simulink model "nape_speed_brakes"  (R2024b)
settings: Solver=VariableStepAuto  StartTime=0.0  StopTime=t_fin  RelTol=1e-3
InitFcn:
  | setup_speed_brakes
values from neighbouring files (symbols this model uses):
  alpha0L = convang(-2.9,'deg','rad')    [setup_speed_brakes.m]
  alphabMax = convang(8.0,'deg','rad')    [setup_speed_brakes.m]
  CD0 = 0.020    (= 0.02)    [setup_speed_brakes.m]
  delta0 = convang(0.0,'deg','rad')    [setup_speed_brakes.m]
  deltac = convang(15,'deg','rad')    [setup_speed_brakes.m]
  deltac2 = convang(15,'deg','rad')    [setup_speed_brakes.m]
  deltac3 = convang(0,'deg','rad')    [setup_speed_brakes.m]
  deltac4 = convang(0,'deg','rad')    [setup_speed_brakes.m]
  g = 9.81    [setup_speed_brakes.m]
  gamma0 = convang(0.0,'deg','rad')    [setup_speed_brakes.m]
  gammac = convang(5,'deg','rad')    [setup_speed_brakes.m]
  gammac2 = convang(0,'deg','rad')    [setup_speed_brakes.m]
  gammac3 = convang(-5,'deg','rad')    [setup_speed_brakes.m]
  gammac4 = convang(0,'deg','rad')    [setup_speed_brakes.m]
  h0 = 3048    [setup_speed_brakes.m]
  kD1 = 2/(S*pi*AReffective)    (= 0.000338404785343)    [setup_speed_brakes.m]
  kL = 2/(S*CLalpha)    (= 0.0012483552919)    [setup_speed_brakes.m]
  kLI = 0.010    (= 0.01)    [setup_speed_brakes.m]
  kLP = 0.50    (= 0.5)    [setup_speed_brakes.m]
  kLSB = -0.00008    (= -8e-05)    [setup_speed_brakes.m]
  knu = 0.075    [setup_speed_brakes.m]
  kSB = -0.00008    (= -8e-05)    [setup_speed_brakes.m]
  kTI = 0.0020    (= 0.002)    [setup_speed_brakes.m]
  kTP = 0.080    (= 0.08)    [setup_speed_brakes.m]
  kWdot = 1.31*1e-5    (= 1.31e-05)    [setup_speed_brakes.m]
  L0 = weight0*cos(gamma0)*cos(nu0)    [setup_speed_brakes.m]
  mass0 = massNom    (= 129003)    [setup_speed_brakes.m]
  nu0 = convang(0.0,'deg','rad')    [setup_speed_brakes.m]
  pL = 2.50    (= 2.5)    [setup_speed_brakes.m]
  pnu = 1.00    (= 1)    [setup_speed_brakes.m]
  pT = 2.00    (= 2)    [setup_speed_brakes.m]
  S = 279.6    [setup_speed_brakes.m]
  SB_AlphaFactorMax = 4    [setup_speed_brakes.m]
  SB_AlphaGain = 0.01    [setup_speed_brakes.m]
  SB_DragFactorMax = 1.5    [setup_speed_brakes.m]
  T0 = D0 + weight0*sin(gamma0)    [setup_speed_brakes.m]
  tc = 5    [setup_speed_brakes.m]
  tc2 = 90    [setup_speed_brakes.m]
  tc3 = 150    [setup_speed_brakes.m]
  tc4 = 240    [setup_speed_brakes.m]
  TMax = 320272    [setup_speed_brakes.m]
  V0 = 178.8    [setup_speed_brakes.m]
  Vc = convvel(450,'mph','m/s')    [setup_speed_brakes.m]
  Vc2 = convvel(420,'mph','m/s')    [setup_speed_brakes.m]
  Vc3 = convvel(400,'mph','m/s')    [setup_speed_brakes.m]
  Vc4 = convvel(400,'mph','m/s')    [setup_speed_brakes.m]
  weightMax = massMax*g    (= 1454567.94)    [setup_speed_brakes.m]
  wind_x = wind(1)    [setup_speed_brakes.m]
  wind_y = wind(2)    [setup_speed_brakes.m]
  wind_z = wind(3)    [setup_speed_brakes.m]
  xEG_0 = 0    [setup_speed_brakes.m]
  yEG_0 = 0    [setup_speed_brakes.m]
libraries: simulink x2, aerolibatmos2 x1
Description:
  | Ricostruzione dal modello clean e dalle figure dell'elaborato. Gli spoiler aumentano CD0 e l'alpha richiesta per la stessa L. La correzione alpha non sottrae direttamente portanza alle EOM.
settings Model: Creator=Aerospace Engineer  LastModifiedBy=vince
settings SolverCC: AlgebraicLoopSolver=TrustRegion
settings DebuggingCC: UnconnectedInputMsg=warning  UnconnectedOutputMsg=warning  UnconnectedLineMsg=warning
settings ModelReferenceCC: EnableRefExpFcnMdlSchedulingChecks=on
settings RTWCC: GPUComputeCapability=3.5  DLArmComputeVersion=19.05

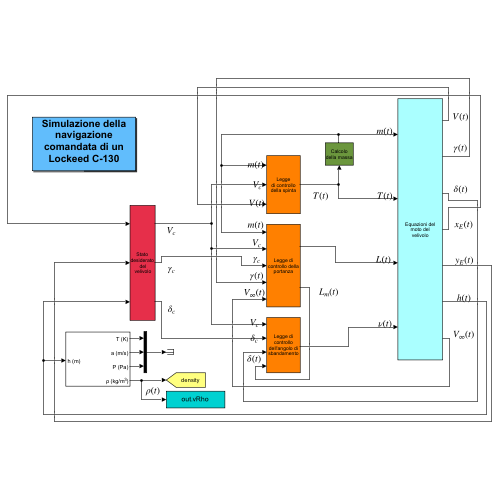
[thumbnail: Simulink's stored preview of the top-level diagram]
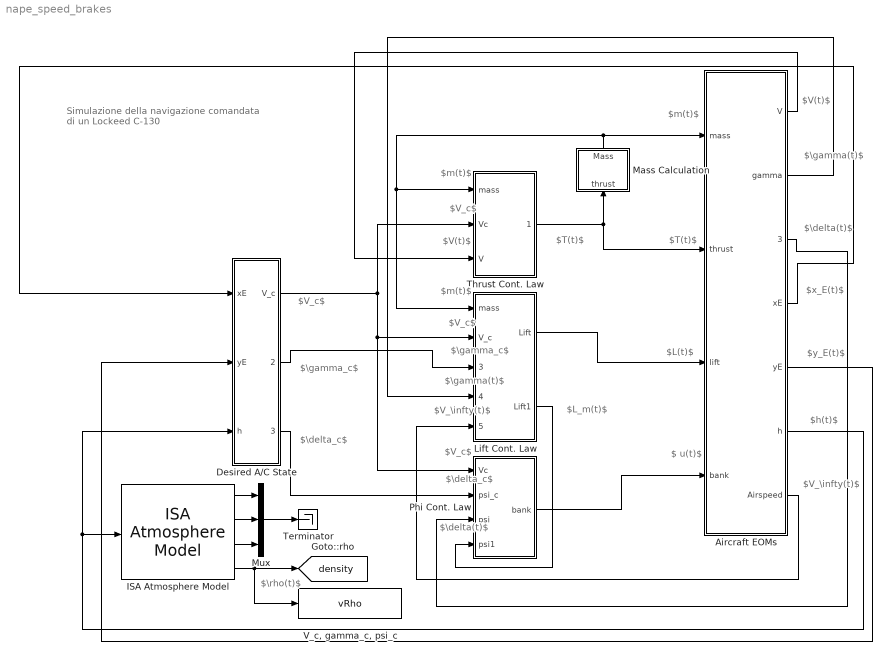
== system nape_speed_brakes ==
  note: $V_\infty(t)$
  note: $m(t)$
  note: Simulazione della navigazione comandata di un Lockeed C-130
  note: $V_c$
  note: $\gamma_c$
  note: $\delta_c$
  note: $V_c$
  note: $V(t)$
  note: $m(t)$
  note: $T(t)$
  note: $T(t)$
  note: $m(t)$
  note: $V_c$
  note: $\gamma_c$
  note: $\gamma(t)$
  note: $V_c$
  note: $\delta_c$
  note: $\delta(t)$
  note: $L(t)$
  note: $\nu(t)$
  note: $V(t)$
  note: $\gamma(t)$
  note: $\delta(t)$
  note: $V_\infty(t)$
  note: $x_E(t)$
  note: $y_E(t)$
  note: $h(t)$
  note: $\rho(t)$
  note: $L_m(t)$
  Aircraft EOMs : Subsystem
      mask Display: disp('Equazioni del\nmoto del\nvelivolo')
  Desired A/C State : Subsystem
      mask Display: disp('Stato\ndesiderato\n del\n velivolo')
  ISA Atmosphere Model : aerolibatmos2/ISA Atmosphere Model  useExtended=off  action=Warning  custom=off  viscosityOut=off  g=9.80665  gamma=1.4  R=287.0531  L=0.0065  h_trop=11000  h_strat=20000  rho0=1.225  P0=101325  T0=288.15  h0=0  S=110.4  Tref=273.15  muref=1.716e-5
  Lift Cont. Law : Subsystem
      mask Display: disp('Legge di\ncontrollo della\nportanza')
  Mass Calculation : Subsystem
      settings: PortSchema="{\"entries\":[{\"content\":{\"sides\":[{\"content\":{\"connectorIds\":[]},\"type\":\"ConnectorPlacement.EquallySpacedRectSide\",\"uuid\":\"6cdda370-62a0-4ac7-b8e8-ad82c4b6b1db\"},{\"content\":{\"connectorIds\":[],\"side\":\"RIGHT\"},\"type\":\"ConnectorPlacement.EquallySpacedRectSide\",\"uuid\":\"1b541650-629f-4986-ba7b-7e8ac2f524da\"},{\"content\":{\"connectorIds\":[\"Out1\"],\"side\":\"TOP\"},\"type\":\"ConnectorPlacement.EquallySpacedRectSide\",\"uuid\":\"ea4f6ba7-6e24-4568-ab7c-c55c2c02c634\"},{\"content\":{\"connectorIds\":[\"In1\"],\"side\":\"BOTTOM\"},\"type\":\"ConnectorPlacement.EquallySpacedRectSide\",\"uuid\":\"57958ebf-54e5-4e2d-a78d-9c6c7d1a65c9\"},{\"content\":{\"connectorIds\":[],\"side\":\"HIDDEN\"},\"type\":\"ConnectorPlacement.EquallySpacedRectSide\",\"uuid\":\"79f4a65c-0d62-441e-9eef-cf8860627e78\"}]},\"type\":\"ConnectorPlacement.EquallySpacedConnector\",\"uuid\":\"ea48c54d-d25b-4ddc-942b-4f525b31fd78\"}],\"packageUris\":[\"http://schema.mathworks.com/mf0/Connector/R2020b\"],\"version\":\"1.0\"}"
      mask Display: disp('Calcolo\ndella massa')
  Mux : Mux  Inputs=3
  Phi Cont. Law : Subsystem
      mask Display: disp('Legge di\ncontrollo\ndell''angolo di\nsbandamento')
  Terminator : Terminator
  Thrust Cont. Law : Subsystem
      mask Display: disp('Legge\ndi controllo\ndella spinta')
  "V_c, gamma_c, psi_c" : ToWorkspace  VariableName=vRho  SaveFormat=Timeseries  SampleTime=-1
  tag scope: density=global
  wires:
  Mux/1 -> Terminator/1
  ISA Atmosphere Model/3 -> Mux/3
  ISA Atmosphere Model/2 -> Mux/2
  ISA Atmosphere Model/1 -> Mux/1
  Desired A/C State/1(V_c) -> Phi Cont. Law/1(Vc), Lift Cont. Law/2(V_c), Thrust Cont. Law/2(Vc)
  Mass Calculation/1("Mass ") -> Lift Cont. Law/1(mass), Thrust Cont. Law/1(mass), Aircraft EOMs/1("mass ")
  Thrust Cont. Law/1(Thrust) -> Aircraft EOMs/2("thrust "), Mass Calculation/1(thrust)
  Desired A/C State/2(gamma_c) -> Lift Cont. Law/3(gamma_c)
  Desired A/C State/3(psi_c) -> Phi Cont. Law/2(psi_c)
  Lift Cont. Law/1(Lift) -> Aircraft EOMs/3("lift ")
  Phi Cont. Law/1(bank) -> Aircraft EOMs/4(bank)
  Aircraft EOMs/1(" V ") -> Thrust Cont. Law/3(V)
  Aircraft EOMs/2(" gamma ") -> Lift Cont. Law/4(gamma)
  Aircraft EOMs/3("  ") -> Phi Cont. Law/3(psi)
  Aircraft EOMs/7(Airspeed) -> Lift Cont. Law/5(Airspeed)
  Aircraft EOMs/4(xE) -> Desired A/C State/1(xE)
  Aircraft EOMs/5(yE) -> Desired A/C State/2(yE)
  Aircraft EOMs/6(h) -> Desired A/C State/3(h), ISA Atmosphere Model/1
  ISA Atmosphere Model/4 -> "V_c, gamma_c, psi_c"/1, [density]
  Lift Cont. Law/2(Lift1) -> Phi Cont. Law/4(psi1)

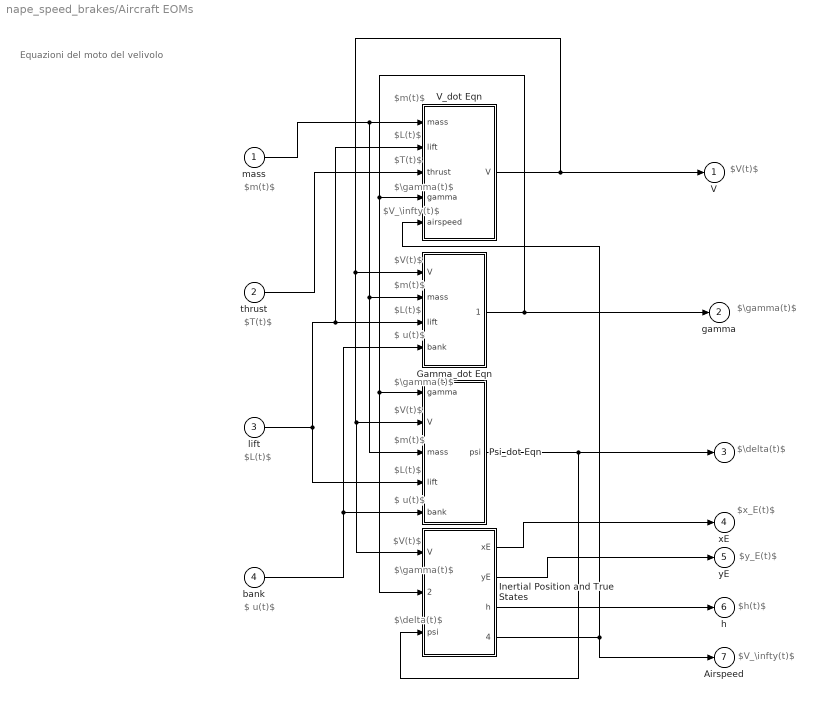
== system nape_speed_brakes/Aircraft EOMs ==
  note: Equazioni del moto
      | del velivolo
  note: $m(t)$
  note: $T(t)$
  note: $L(t)$
  note: $\nu(t)$
  note: $V(t)$
  note: $m(t)$
  note: $L(t)$
  note: $T(t)$
  note: $V(t)$
  note: $m(t)$
  note: $L(t)$
  note: $\nu(t)$
  note: $\gamma(t)$
  note: $\gamma(t)$
  note: $\gamma(t)$
  note: $V(t)$
  note: $m(t)$
  note: $L(t)$
  note: $\nu(t)$
  note: $\delta(t)$
  note: $V(t)$
  note: $\gamma(t)$
  note: $\delta(t)$
  note: $x_E(t)$
  note: $y_E(t)$
  note: $h(t)$
  note: $V_\infty(t)$
  note: $V_\infty(t)$
  "mass " : Inport
  "thrust " : Inport  Port=2
  "lift " : Inport  Port=3
  bank : Inport  Port=4
  Gamma_dot Eqn : Subsystem
      mask Display: disp('Equazione \ndell''angolo\n di rampa')
  Inertial Position and True States : Subsystem
      mask Display: disp('Coordinate\ndel baricentro\ne corrente\n relativa')
  Psi_dot Eqn : Subsystem
      mask Display: disp('Equazione\ndell''angolo\n di virata')
  V_dot Eqn : Subsystem
      mask Display: disp('Equazione \n della velocità')
  " V " : Outport
  " gamma " : Outport  Port=2
  "  " : Outport  Port=3
  xE : Outport  Port=4
  yE : Outport  Port=5
  h : Outport  Port=6
  Airspeed : Outport  Port=7
  wires:
  "mass "/1 -> Psi_dot Eqn/3(mass), Gamma_dot Eqn/2(mass), V_dot Eqn/1(mass)
  "lift "/1 -> Gamma_dot Eqn/3("lift "), V_dot Eqn/2(lift), Psi_dot Eqn/4("lift ")
  "thrust "/1 -> V_dot Eqn/3(thrust)
  V_dot Eqn/1(V) -> Inertial Position and True States/1(V), Psi_dot Eqn/2(V), Gamma_dot Eqn/1(V), " V "/1
  bank/1 -> Psi_dot Eqn/5(bank), Gamma_dot Eqn/4(bank)
  Gamma_dot Eqn/1(Gamma) -> " gamma "/1, Inertial Position and True States/2("gamma "), Psi_dot Eqn/1(gamma), V_dot Eqn/4(gamma)
  Psi_dot Eqn/1(psi) -> Inertial Position and True States/3(psi), "  "/1
  Inertial Position and True States/1(xE) -> xE/1
  Inertial Position and True States/2(yE) -> yE/1
  Inertial Position and True States/3(h) -> h/1
  Inertial Position and True States/4(AirSpeed) -> Airspeed/1, V_dot Eqn/5(airspeed)

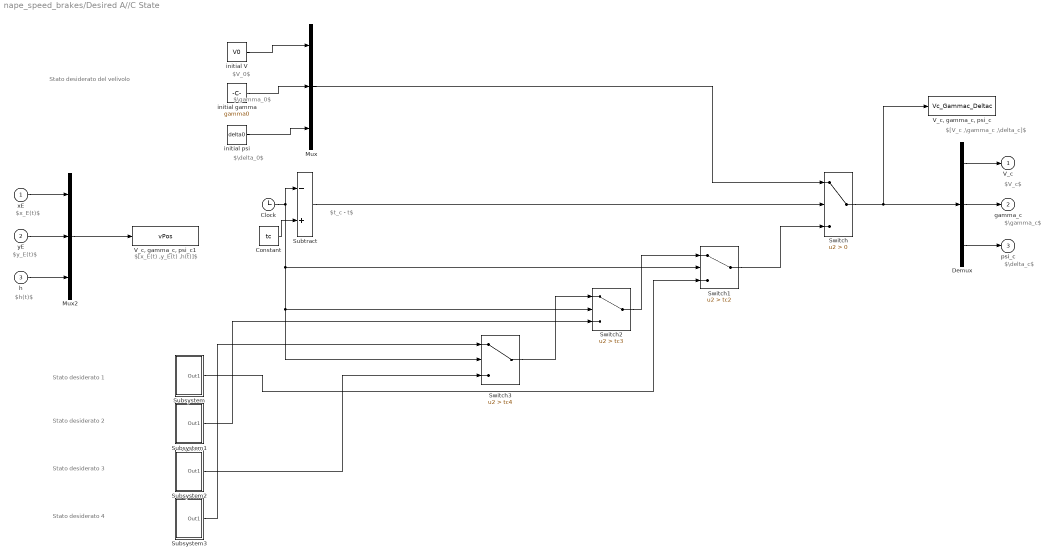
== system nape_speed_brakes/Desired A//C State ==
  note: $[V_c ,\gamma_c ,\delta_c]$
  note: $t_c - t$
  note: $\delta_0$
  note: $\gamma_0$
  note: $V_0$
  note: Stato desiderato
      | del velivolo
  note: $V_c$
  note: $\gamma_c$
  note: $\delta_c$
  note: $x_E(t)$
  note: $h(t)$
  note: $y_E(t)$
  note: $[x_E(t) ,y_E(t) ,h(t)]$
  note: Stato desiderato 1
  note: Stato desiderato 2
  note: Stato desiderato 3
  note: Stato desiderato 4
  xE : Inport
  yE : Inport  Port=2
  h : Inport  Port=3
  Clock : Clock
  Constant : Constant  Value=tc
  Demux : Demux  Outputs=3
  Mux : Mux  Inputs=3
  Mux2 : Mux  Inputs=3
  Subsystem : Subsystem
  Subsystem1 : Subsystem
  Subsystem2 : Subsystem
  Subsystem3 : Subsystem
  Subtract : Sum  Inputs=-+
  Switch : Switch  Criteria=u2 > Threshold  SaturateOnIntegerOverflow=off  InputSameDT=off
  Switch1 : Switch  Criteria=u2 > Threshold  Threshold=tc2  SaturateOnIntegerOverflow=off  InputSameDT=off
  Switch2 : Switch  Criteria=u2 > Threshold  Threshold=tc3  SaturateOnIntegerOverflow=off  InputSameDT=off
  Switch3 : Switch  Criteria=u2 > Threshold  Threshold=tc4  SaturateOnIntegerOverflow=off  InputSameDT=off
  "V_c, gamma_c, psi_c" : ToWorkspace  VariableName=Vc_Gammac_Deltac  SaveFormat=Timeseries  SampleTime=-1
  "V_c, gamma_c, psi_c1" : ToWorkspace  VariableName=vPos  SaveFormat=Timeseries  SampleTime=-1
  initial V : Constant  Value=V0
  initial gamma : Constant  Value=gamma0
  initial psi : Constant  Value=delta0
  V_c : Outport
  gamma_c : Outport  Port=2
  psi_c : Outport  Port=3
  wires:
  xE/1 -> Mux2/1
  yE/1 -> Mux2/2
  h/1 -> Mux2/3
  Constant/1 -> Subtract/2
  Clock/1 -> Switch3/2, Switch2/2, Switch1/2, Subtract/1
  initial gamma/1 -> Mux/2
  initial V/1 -> Mux/1
  initial psi/1 -> Mux/3
  Mux/1 -> Switch/1
  Subtract/1 -> Switch/2
  Switch/1 -> "V_c, gamma_c, psi_c"/1, Demux/1
  Demux/1 -> V_c/1
  Demux/2 -> gamma_c/1
  Demux/3 -> psi_c/1
  Mux2/1 -> "V_c, gamma_c, psi_c1"/1
  Switch1/1 -> Switch/3
  Switch3/1 -> Switch2/1
  Switch2/1 -> Switch1/1
  Subsystem/1(Out1) -> Switch1/3
  Subsystem1/1(Out1) -> Switch2/3
  Subsystem2/1(Out1) -> Switch3/3
  Subsystem3/1(Out1) -> Switch3/1

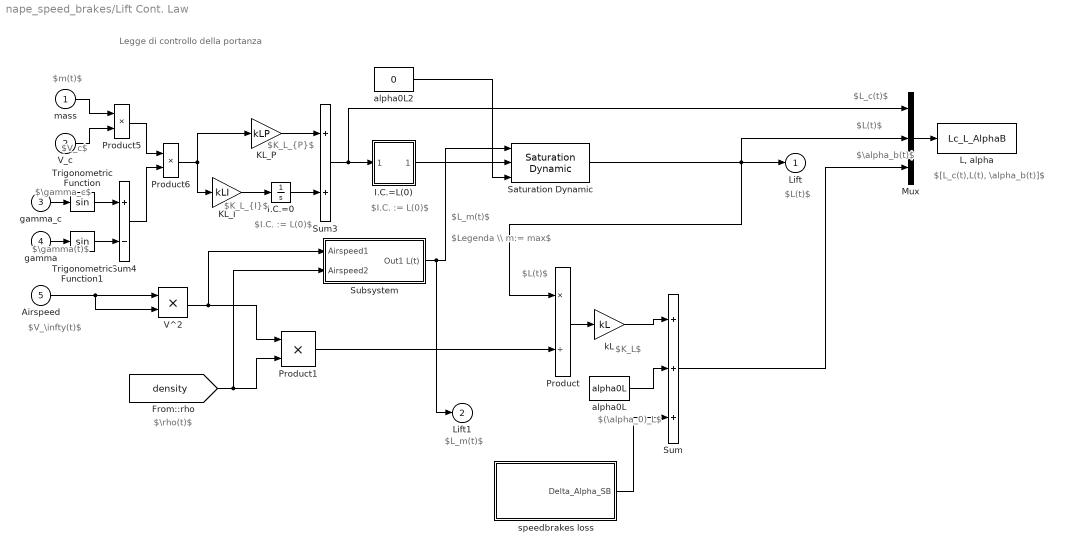
== system nape_speed_brakes/Lift Cont. Law ==
  note: $[L_c(t),L(t), \alpha_b(t)]$
  note: $K_L$
  note: $m(t)$
  note: $V_c$
  note: $\gamma_c$
  note: $\gamma(t)$
  note: $V_\infty(t)$
  note: Legge di controllo
      | della portanza
  note: $K_L_{P}$
  note: $K_L_{I}$
  note: $I.C. := L(0)$
  note: $L_c(t)$
  note: $I.C. := L(0)$
  note: $L_m(t)$
  note: $Legenda \\ m:= max$
  note: $L(t)$
  note: $L(t)$
  note: $L(t)$
  note: $\rho(t)$
  note: $(\alpha_0)_L$
  note: $\alpha_b(t)$
  note: $L_m(t)$
  mass : Inport
  V_c : Inport  Port=2
  gamma_c : Inport  Port=3
  gamma : Inport  Port=4
  Airspeed : Inport  Port=5
  I.C.=0 : Integrator  InitialCondition=L0
  I.C.=L(0) : Subsystem
      mask Display: disp('pL\n-----\ns + pL')
  KL_I : Gain  Gain=kLI  SaturateOnIntegerOverflow=on  OutDataTypeStr=Inherit: Same as input  ParamDataTypeStr=Inherit: Same as input
  KL_P : Gain  Gain=kLP  SaturateOnIntegerOverflow=on  OutDataTypeStr=Inherit: Same as input  ParamDataTypeStr=Inherit: Same as input
  "L, alpha" : ToWorkspace  VariableName=Lc_L_AlphaB  SaveFormat=Timeseries  SampleTime=-1
  Mux : Mux  Inputs=3
  Product : Product  Inputs=*/
  Product1 : Product  InputSameDT=on  RndMeth=Zero  SaturateOnIntegerOverflow=on  OutDataTypeStr=Inherit: Same as first input
  Product5 : Product  InputSameDT=on  RndMeth=Zero  SaturateOnIntegerOverflow=on  OutDataTypeStr=Inherit: Same as first input
  Product6 : Product  InputSameDT=on  RndMeth=Zero  SaturateOnIntegerOverflow=on  OutDataTypeStr=Inherit: Same as first input
  Saturation Dynamic : simulink/Discontinuities/Saturation Dynamic  OutMin=[]  OutMax=[]  OutDataTypeStr=Inherit: Same as second input  OutDataType=fixdt(1, 16)  OutScaling=2^-10  DoSatur=off
  Subsystem : Subsystem
  Sum : Sum  Inputs=+++  InputSameDT=on  SaturateOnIntegerOverflow=on  OutDataTypeStr=Inherit: Same as first input
  Sum3 : Sum  InputSameDT=on  SaturateOnIntegerOverflow=on  OutDataTypeStr=Inherit: Same as first input
  Sum4 : Sum  Inputs=+-  InputSameDT=on  SaturateOnIntegerOverflow=on  OutDataTypeStr=Inherit: Same as first input
  Trigonometric Function : Trigonometry
  Trigonometric Function1 : Trigonometry
  V^2 : Product  InputSameDT=on  RndMeth=Zero  SaturateOnIntegerOverflow=on  OutDataTypeStr=Inherit: Same as first input
  alpha0L : Constant  Value=alpha0L
  alpha0L2 : Constant  Value=0
  kL : Gain  Gain=kL  SaturateOnIntegerOverflow=on  OutDataTypeStr=Inherit: Same as input  ParamDataTypeStr=Inherit: Same as input
  speedbrakes loss : Subsystem
  Lift : Outport
  Lift1 : Outport  Port=2
  wires:
  Sum3/1 -> I.C.=L(0)/1(In1 Lc(t)), Mux/1
  Sum4/1 -> Product6/2
  V_c/1 -> Product5/2
  mass/1 -> Product5/1
  Product5/1 -> Product6/1
  KL_P/1 -> Sum3/1
  I.C.=0/1 -> Sum3/2
  KL_I/1 -> I.C.=0/1
  Airspeed/1 -> V^2/1, V^2/2
  Product/1 -> kL/1
  kL/1 -> Sum/1
  Sum/1 -> Mux/3
  alpha0L/1 -> Sum/2
  V^2/1 -> Subsystem/1(Airspeed1), Product1/1
  [density] -> Subsystem/2(Airspeed2), Product1/2
  Product1/1 -> Product/2
  Mux/1 -> "L, alpha"/1
  gamma_c/1 -> Trigonometric Function/1
  Trigonometric Function/1 -> Sum4/1
  gamma/1 -> Trigonometric Function1/1
  Trigonometric Function1/1 -> Sum4/2
  Product6/1 -> KL_I/1, KL_P/1
  I.C.=L(0)/1(Out1 L(t)) -> Saturation Dynamic/2
  Subsystem/1(Out1 L(t)) -> Lift1/1, Saturation Dynamic/1
  alpha0L2/1 -> Saturation Dynamic/3
  Saturation Dynamic/1 -> Mux/2, Lift/1, Product/1
  speedbrakes loss/1(Delta_Alpha_SB) -> Sum/3

== system nape_speed_brakes/Mass Calculation ==
  note: $\dot{m}(t)$
  note: $-K_\dot{W}$
  note: $T(t)$
  note: $I.C. := m(0)$
  note: $m(t)$
  note: $m(t)$
  note: Calcolo della massa
  thrust : Inport
  -Kwdot : Gain  Gain=-kWdot  SaturateOnIntegerOverflow=on  OutDataTypeStr=Inherit: Same as input  ParamDataTypeStr=Inherit: Same as input
  I.C. = mass(0) : Integrator  InitialCondition=mass0
  To Workspace : ToWorkspace  VariableName=vMass  SaveFormat=Timeseries  SampleTime=-1
  "Mass " : Outport
  wires:
  -Kwdot/1 -> I.C. = mass(0)/1
  I.C. = mass(0)/1 -> To Workspace/1, "Mass "/1
  thrust/1 -> -Kwdot/1

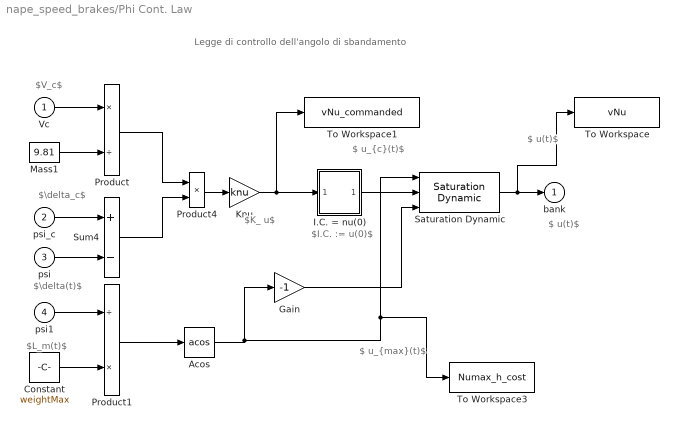
== system nape_speed_brakes/Phi Cont. Law ==
  note: Legge di controllo
      | dell'angolo di sbandamento
  note: $V_c$
  note: $\delta_c$
  note: $\delta(t)$
  note: $K_\nu$
  note: $I.C. := \nu(0)$
  note: $\nu(t)$
  note: $\nu(t)$
  note: $\nu_{c}(t)$
  note: $L_m(t)$
  note: $\nu_{max}(t)$
  Vc : Inport
  psi_c : Inport  Port=2
  psi : Inport  Port=3
  psi1 : Inport  Port=4
  Acos : Trigonometry  Operator=acos
  Constant : Constant  Value=weightMax
  Gain : Gain  Gain=-1
  I.C. = nu(0) : Subsystem
      mask Display: disp('pf\n-----\ns + pf')
  Knu : Gain  Gain=knu  SaturateOnIntegerOverflow=on  OutDataTypeStr=Inherit: Same as input  ParamDataTypeStr=Inherit: Same as input
  Mass1 : Constant  Value=9.81
  Product : Product  Inputs=*/
  Product1 : Product  Inputs=/*
  Product4 : Product  InputSameDT=on  RndMeth=Zero  SaturateOnIntegerOverflow=on  OutDataTypeStr=Inherit: Same as first input
  Saturation Dynamic : simulink/Discontinuities/Saturation Dynamic  OutMin=[]  OutMax=[]  OutDataTypeStr=Inherit: Same as second input  OutDataType=fixdt(1, 16)  OutScaling=2^-10  DoSatur=off
  Sum4 : Sum  Inputs=+-  InputSameDT=on  SaturateOnIntegerOverflow=on  OutDataTypeStr=Inherit: Same as first input
  To Workspace : ToWorkspace  VariableName=vNu  SaveFormat=Timeseries  SampleTime=-1
  To Workspace1 : ToWorkspace  VariableName=vNu_commanded  SaveFormat=Timeseries  SampleTime=-1
  To Workspace3 : ToWorkspace  VariableName=Numax_h_cost  SaveFormat=Timeseries  SampleTime=-1
  bank : Outport
  wires:
  Knu/1 -> To Workspace1/1, I.C. = nu(0)/1(In1 nu_c)
  Product4/1 -> Knu/1
  psi/1 -> Sum4/2
  psi_c/1 -> Sum4/1
  Sum4/1 -> Product4/2
  Vc/1 -> Product/1
  Mass1/1 -> Product/2
  Product/1 -> Product4/1
  Constant/1 -> Product1/2
  psi1/1 -> Product1/1
  Product1/1 -> Acos/1
  I.C. = nu(0)/1(Out1 nu) -> Saturation Dynamic/2
  Acos/1 -> To Workspace3/1, Saturation Dynamic/1, Gain/1
  Gain/1 -> Saturation Dynamic/3
  Saturation Dynamic/1 -> To Workspace/1, bank/1

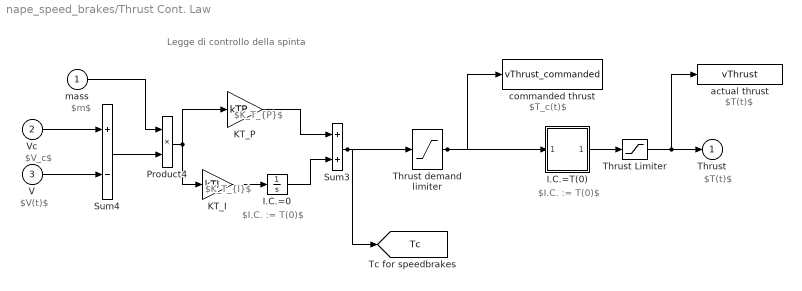
== system nape_speed_brakes/Thrust Cont. Law ==
  note: $T_c(t)$
  note: $I.C. := T(0)$
  note: $K_T_{P}$
  note: $V(t)$
  note: $m$
  note: Legge di controllo
      | della spinta
  note: $V_c$
  note: $K_T_{I}$
  note: $I.C. := T(0)$
  note: $T(t)$
  note: $T(t)$
  mass : Inport
  Vc : Inport  Port=2
  V : Inport  Port=3
  I.C.=0 : Integrator  InitialCondition=T0
  I.C.=T(0) : Subsystem
      mask Display: disp('pT\n-----\ns + pT')
  KT_I : Gain  Gain=kTI  SaturateOnIntegerOverflow=on  OutDataTypeStr=Inherit: Same as input  ParamDataTypeStr=Inherit: Same as input
  KT_P : Gain  Gain=kTP  SaturateOnIntegerOverflow=on  OutDataTypeStr=Inherit: Same as input  ParamDataTypeStr=Inherit: Same as input
  Product4 : Product  InputSameDT=on  RndMeth=Zero  SaturateOnIntegerOverflow=on  OutDataTypeStr=Inherit: Same as first input
  Sum3 : Sum  InputSameDT=on  SaturateOnIntegerOverflow=on  OutDataTypeStr=Inherit: Same as first input
  Sum4 : Sum  Inputs=+-  InputSameDT=on  SaturateOnIntegerOverflow=on  OutDataTypeStr=Inherit: Same as first input
  Thrust Limiter : Saturate  UpperLimit=TMax  LowerLimit=0
  Thrust demand limiter : Saturate  UpperLimit=TMax  LowerLimit=0
  actual thrust : ToWorkspace  VariableName=vThrust  SaveFormat=Timeseries  SampleTime=-1
  commanded thrust : ToWorkspace  VariableName=vThrust_commanded  SaveFormat=Timeseries  SampleTime=-1
  Thrust : Outport
  tag scope: Tc=global
  wires:
  Thrust Limiter/1 -> Thrust/1, actual thrust/1
  I.C.=T(0)/1(Out1 T(t)) -> Thrust Limiter/1
  Product4/1 -> KT_P/1, KT_I/1
  V/1 -> Sum4/2
  Vc/1 -> Sum4/1
  KT_P/1 -> Sum3/1
  KT_I/1 -> I.C.=0/1
  mass/1 -> Product4/1
  Sum3/1 -> [Tc], Thrust demand limiter/1
  I.C.=0/1 -> Sum3/2
  Sum4/1 -> Product4/2
  Thrust demand limiter/1 -> I.C.=T(0)/1(In1 Tc(t)), commanded thrust/1

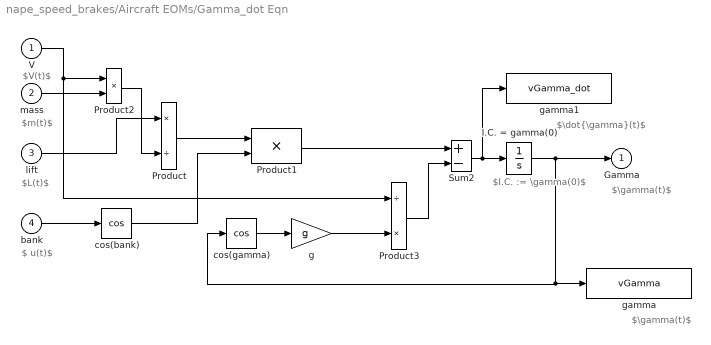
== system nape_speed_brakes/Aircraft EOMs/Gamma_dot Eqn ==
  note: $V(t)$
  note: $m(t)$
  note: $L(t)$
  note: $\nu(t)$
  note: $I.C. := \gamma(0)$
  note: $\gamma(t)$
  note: $\gamma(t)$
  note: $\dot{\gamma}(t)$
  V : Inport
  mass : Inport  Port=2
  "lift " : Inport  Port=3
  bank : Inport  Port=4
  I.C. = gamma(0) : Integrator  InitialCondition=gamma0
  Product : Product  Inputs=*/
  Product1 : Product  InputSameDT=on  RndMeth=Zero  SaturateOnIntegerOverflow=on  OutDataTypeStr=Inherit: Same as first input
  Product2 : Product  InputSameDT=on  RndMeth=Zero  SaturateOnIntegerOverflow=on  OutDataTypeStr=Inherit: Same as first input
  Product3 : Product  Inputs=/*
  Sum2 : Sum  Inputs=+-  InputSameDT=on  SaturateOnIntegerOverflow=on  OutDataTypeStr=Inherit: Same as first input
  cos(bank) : Trigonometry  Operator=cos
  cos(gamma) : Trigonometry  Operator=cos
  g : Gain  Gain=g
  gamma : ToWorkspace  VariableName=vGamma  SaveFormat=Timeseries  SampleTime=-1
  gamma1 : ToWorkspace  VariableName=vGamma_dot  SaveFormat=Timeseries  SampleTime=-1
  Gamma : Outport
  wires:
  cos(bank)/1 -> Product1/2
  bank/1 -> cos(bank)/1
  "lift "/1 -> Product/1
  mass/1 -> Product2/2
  V/1 -> Product3/1, Product2/1
  Sum2/1 -> gamma1/1, I.C. = gamma(0)/1
  cos(gamma)/1 -> g/1
  Product1/1 -> Sum2/1
  Product/1 -> Product1/1
  Product2/1 -> Product/2
  Product3/1 -> Sum2/2
  g/1 -> Product3/2
  I.C. = gamma(0)/1 -> Gamma/1, gamma/1, cos(gamma)/1

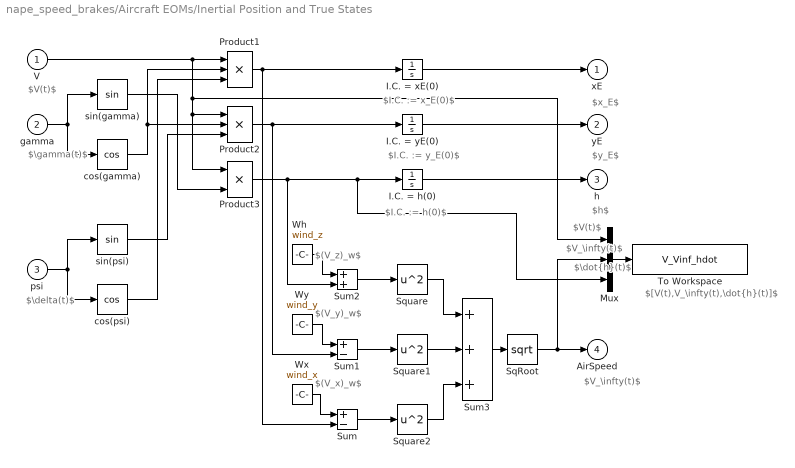
== system nape_speed_brakes/Aircraft EOMs/Inertial Position and True States ==
  note: $[V(t),V_\infty(t),\dot{h}(t)]$
  note: $\dot{h}(t)$
  note: $(V_z)_w$
  note: $x_E$
  note: $\delta(t)$
  note: $V(t)$
  note: $\gamma(t)$
  note: $I.C. := x_E(0)$
  note: $I.C. := y_E(0)$
  note: $I.C. := h(0)$
  note: $y_E$
  note: $h$
  note: $(V_y)_w$
  note: $(V_x)_w$
  note: $V(t)$
  note: $V_\infty(t)$
  note: $V_\infty(t)$
  V : Inport
  "gamma " : Inport  Port=2
  psi : Inport  Port=3
  I.C. = h(0) : Integrator  InitialCondition=h0
  I.C. = xE(0) : Integrator  InitialCondition=xEG_0
  I.C. = yE(0) : Integrator  InitialCondition=yEG_0
  Mux : Mux  Inputs=3
  Product1 : Product  Inputs=3  InputSameDT=on  RndMeth=Zero  SaturateOnIntegerOverflow=on  OutDataTypeStr=Inherit: Same as first input
  Product2 : Product  Inputs=3  InputSameDT=on  RndMeth=Zero  SaturateOnIntegerOverflow=on  OutDataTypeStr=Inherit: Same as first input
  Product3 : Product  InputSameDT=on  RndMeth=Zero  SaturateOnIntegerOverflow=on  OutDataTypeStr=Inherit: Same as first input
  SqRoot : Math  Operator=sqrt  SignedPower=on
  Square : Math  Operator=square  SignedPower=on
  Square1 : Math  Operator=square  SignedPower=on
  Square2 : Math  Operator=square  SignedPower=on
  Sum : Sum  Inputs=+-  InputSameDT=on  SaturateOnIntegerOverflow=on  OutDataTypeStr=Inherit: Same as first input
  Sum1 : Sum  Inputs=+-  InputSameDT=on  SaturateOnIntegerOverflow=on  OutDataTypeStr=Inherit: Same as first input
  Sum2 : Sum  InputSameDT=on  SaturateOnIntegerOverflow=on  OutDataTypeStr=Inherit: Same as first input
  Sum3 : Sum  Inputs=+++  InputSameDT=on  SaturateOnIntegerOverflow=on  OutDataTypeStr=Inherit: Same as first input
  To Workspace : ToWorkspace  VariableName=V_Vinf_hdot  SaveFormat=Timeseries  SampleTime=-1
  Wh : Constant  Value=wind_z
  Wx : Constant  Value=wind_x
  Wy : Constant  Value=wind_y
  cos(gamma) : Trigonometry  Operator=cos
  cos(psi) : Trigonometry  Operator=cos
  sin(gamma) : Trigonometry
  sin(psi) : Trigonometry
  xE : Outport
  yE : Outport  Port=2
  h : Outport  Port=3
  AirSpeed : Outport  Port=4
  wires:
  "gamma "/1 -> cos(gamma)/1, sin(gamma)/1
  psi/1 -> sin(psi)/1, cos(psi)/1
  cos(psi)/1 -> Product1/3
  V/1 -> Mux/1, Product2/1, Product3/1, Product1/1
  cos(gamma)/1 -> Product1/2, Product2/2
  sin(psi)/1 -> Product2/3
  sin(gamma)/1 -> Product3/2
  I.C. = xE(0)/1 -> xE/1
  I.C. = yE(0)/1 -> yE/1
  I.C. = h(0)/1 -> h/1
  Product3/1 -> Mux/3, I.C. = h(0)/1, Sum2/2
  Product2/1 -> I.C. = yE(0)/1, Sum1/2
  Product1/1 -> I.C. = xE(0)/1, Sum/2
  Wx/1 -> Sum/1
  Wy/1 -> Sum1/1
  Wh/1 -> Sum2/1
  Sum2/1 -> Square/1
  Sum1/1 -> Square1/1
  Sum/1 -> Square2/1
  Sum3/1 -> SqRoot/1
  SqRoot/1 -> Mux/2, AirSpeed/1
  Square1/1 -> Sum3/2
  Square/1 -> Sum3/1
  Square2/1 -> Sum3/3
  Mux/1 -> To Workspace/1

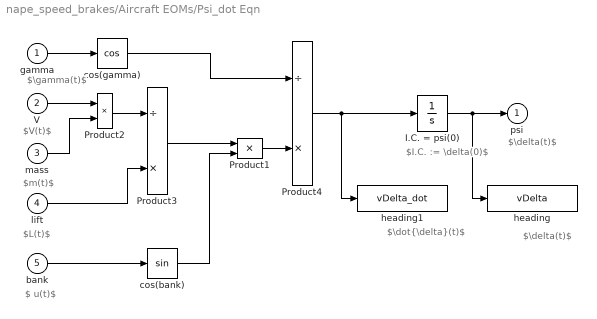
== system nape_speed_brakes/Aircraft EOMs/Psi_dot Eqn ==
  note: $\dot{\delta}(t)$
  note: $\gamma(t)$
  note: $V(t)$
  note: $m(t)$
  note: $L(t)$
  note: $\nu(t)$
  note: $I.C. := \delta(0)$
  note: $\delta(t)$
  note: $\delta(t)$
  gamma : Inport
  V : Inport  Port=2
  mass : Inport  Port=3
  "lift " : Inport  Port=4
  bank : Inport  Port=5
  I.C. = psi(0) : Integrator  InitialCondition=delta0
  Product1 : Product  InputSameDT=on  RndMeth=Zero  SaturateOnIntegerOverflow=on  OutDataTypeStr=Inherit: Same as first input
  Product2 : Product  InputSameDT=on  RndMeth=Zero  SaturateOnIntegerOverflow=on  OutDataTypeStr=Inherit: Same as first input
  Product3 : Product  Inputs=/*  InputSameDT=on  RndMeth=Zero  SaturateOnIntegerOverflow=on  OutDataTypeStr=Inherit: Same as first input
  Product4 : Product  Inputs=/*  InputSameDT=on  RndMeth=Zero  SaturateOnIntegerOverflow=on  OutDataTypeStr=Inherit: Same as first input
  cos(bank) : Trigonometry
  cos(gamma) : Trigonometry  Operator=cos
  heading : ToWorkspace  VariableName=vDelta  SaveFormat=Timeseries  SampleTime=-1
  heading1 : ToWorkspace  VariableName=vDelta_dot  SaveFormat=Timeseries  SampleTime=-1
  psi : Outport
  wires:
  Product4/1 -> heading1/1, I.C. = psi(0)/1
  cos(gamma)/1 -> Product4/1
  gamma/1 -> cos(gamma)/1
  cos(bank)/1 -> Product1/2
  bank/1 -> cos(bank)/1
  I.C. = psi(0)/1 -> heading/1, psi/1
  mass/1 -> Product2/2
  V/1 -> Product2/1
  Product3/1 -> Product1/1
  Product1/1 -> Product4/2
  Product2/1 -> Product3/1
  "lift "/1 -> Product3/2

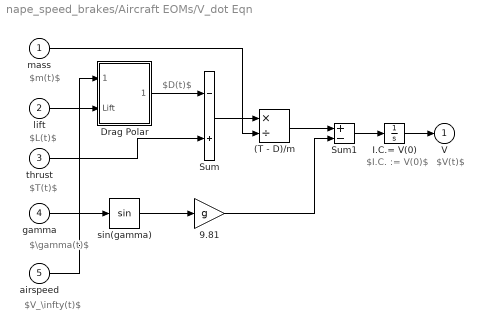
== system nape_speed_brakes/Aircraft EOMs/V_dot Eqn ==
  note: $m(t)$
  note: $L(t)$
  note: $T(t)$
  note: $\gamma(t)$
  note: $V_\infty(t)$
  note: $D(t)$
  note: $V(t)$
  note: $I.C. := V(0)$
  mass : Inport
  lift : Inport  Port=2
  thrust : Inport  Port=3
  gamma : Inport  Port=4
  airspeed : Inport  Port=5
  (T - D)/m : Product  Inputs=*/
  9.81 : Gain  Gain=g
  Drag Polar : Subsystem
      mask Display: disp('Polare\n di\n resistenza\n parabolica')
  I.C.= V(0) : Integrator  InitialCondition=V0
  Sum : Sum  Inputs=-+  InputSameDT=on  SaturateOnIntegerOverflow=on  OutDataTypeStr=Inherit: Same as first input
  Sum1 : Sum  Inputs=+-  InputSameDT=on  SaturateOnIntegerOverflow=on  OutDataTypeStr=Inherit: Same as first input
  sin(gamma) : Trigonometry
  V : Outport
  wires:
  gamma/1 -> sin(gamma)/1
  lift/1 -> Drag Polar/2(Lift)
  sin(gamma)/1 -> 9.81/1
  (T - D)/m/1 -> Sum1/1
  9.81/1 -> Sum1/2
  Sum1/1 -> I.C.= V(0)/1
  I.C.= V(0)/1 -> V/1
  airspeed/1 -> Drag Polar/1(Airspeed)
  thrust/1 -> Sum/2
  Drag Polar/1(Drag) -> Sum/1
  mass/1 -> (T - D)/m/2
  Sum/1 -> (T - D)/m/1

== system nape_speed_brakes/Desired A//C State/Subsystem ==
  note: $\delta_c$
  note: $\gamma_c$
  note: $V_c$
  "Commanded Speed " : Constant  Value=Vc
  Commanded flight path angle : Constant  Value=gammac
  Commanded heading angle : Constant  Value=deltac
  Mux6 : Mux  Inputs=3
  Out1 : Outport
  wires:
  Commanded flight path angle/1 -> Mux6/2
  Commanded heading angle/1 -> Mux6/3
  "Commanded Speed "/1 -> Mux6/1
  Mux6/1 -> Out1/1

== system nape_speed_brakes/Desired A//C State/Subsystem1 ==
  note: $\delta_c$
  note: $V_c$
  note: $\gamma_c$
  Commanded Speed 1 : Constant  Value=Vc2
  Commanded flight path angle1 : Constant  Value=gammac2
  Commanded heading angle1 : Constant  Value=deltac2
  Mux3 : Mux  Inputs=3
  Out1 : Outport
  wires:
  Commanded flight path angle1/1 -> Mux3/2
  Commanded Speed 1/1 -> Mux3/1
  Mux3/1 -> Out1/1
  Commanded heading angle1/1 -> Mux3/3

== system nape_speed_brakes/Desired A//C State/Subsystem2 ==
  note: $V_c$
  note: $\gamma_c$
  note: $\delta_c$
  Commanded Speed 2 : Constant  Value=Vc3
  Commanded flight path angle2 : Constant  Value=gammac3
  Commanded heading angle2 : Constant  Value=deltac3
  Mux4 : Mux  Inputs=3
  Out1 : Outport
  wires:
  Commanded Speed 2/1 -> Mux4/1
  Commanded heading angle2/1 -> Mux4/3
  Commanded flight path angle2/1 -> Mux4/2
  Mux4/1 -> Out1/1

== system nape_speed_brakes/Desired A//C State/Subsystem3 ==
  note: $V_c$
  note: $\gamma_c$
  note: $\delta_c$
  Commanded Speed 3 : Constant  Value=Vc4
  Commanded flight path angle3 : Constant  Value=gammac4
  Commanded heading angle3 : Constant  Value=deltac4
  Mux5 : Mux  Inputs=3
  Out1 : Outport
  wires:
  Commanded Speed 3/1 -> Mux5/1
  Commanded heading angle3/1 -> Mux5/3
  Commanded flight path angle3/1 -> Mux5/2
  Mux5/1 -> Out1/1

== system nape_speed_brakes/Lift Cont. Law/I.C.=L(0) ==
  note: $x(t) = L(t) \\ u(t) = L_c(t)$
  note: $I.C. := L(0)$
  note: $L_c(t)$
  note: $L(t)$
  In1 Lc(t) : Inport
  I.C.=L(0) : StateSpace  A=-pL  B=pL  D=0  InitialCondition=L0
  Out1 L(t) : Outport
  wires:
  In1 Lc(t)/1 -> I.C.=L(0)/1
  I.C.=L(0)/1 -> Out1 L(t)/1

== system nape_speed_brakes/Lift Cont. Law/Subsystem ==
  note: $Legenda \\ m:= max \\ L:= Lift$
  note: $(\alpha_b)_m$
  note: $(\alpha_0)_L$
  note: $L_m(t)$
  note: $\rho(t)$
  note: $V^2_\infty(t)$
  note: $K_L$
  Airspeed1 : Inport
  Airspeed2 : Inport  Port=2
  KL_P1 : Gain  Gain=1/kL  SaturateOnIntegerOverflow=on  OutDataTypeStr=Inherit: Same as input  ParamDataTypeStr=Inherit: Same as input
  Product2 : Product  InputSameDT=on  RndMeth=Zero  SaturateOnIntegerOverflow=on  OutDataTypeStr=Inherit: Same as first input
  Product3 : Product  InputSameDT=on  RndMeth=Zero  SaturateOnIntegerOverflow=on  OutDataTypeStr=Inherit: Same as first input
  Sum1 : Sum  Inputs=+-  InputSameDT=on  SaturateOnIntegerOverflow=on  OutDataTypeStr=Inherit: Same as first input
  alpha0L1 : Constant  Value=alpha0L
  alpha0L2 : Constant  Value=alphabMax
  Out1 L(t) : Outport
  wires:
  alpha0L2/1 -> Sum1/1
  Product2/1 -> Product3/2
  Sum1/1 -> KL_P1/1
  KL_P1/1 -> Product3/1
  alpha0L1/1 -> Sum1/2
  Product3/1 -> Out1 L(t)/1
  Airspeed1/1 -> Product2/1
  Airspeed2/1 -> Product2/2

== system nape_speed_brakes/Lift Cont. Law/speedbrakes loss ==
  Alpha gain : Gain  Gain=SB_AlphaGain
  Deployment limiter : Saturate  UpperLimit=SB_AlphaFactorMax  LowerLimit=1
  KLSB : Gain  Gain=kLSB
  Minus one : Sum  Inputs=+-
  Negative thrust : Switch  Criteria=u2 > Threshold  SaturateOnIntegerOverflow=off  InputSameDT=off
  One : Constant
  Zero : Constant  Value=0
  Delta_Alpha_SB : Outport
  wires:
  [Tc] -> KLSB/1, Negative thrust/2
  KLSB/1 -> Deployment limiter/1
  Deployment limiter/1 -> Minus one/1
  One/1 -> Minus one/2
  Minus one/1 -> Alpha gain/1
  Alpha gain/1 -> Negative thrust/3
  Zero/1 -> Negative thrust/1
  Negative thrust/1 -> Delta_Alpha_SB/1

== system nape_speed_brakes/Phi Cont. Law/I.C. = nu(0) ==
  note: $x(t) = \nu(t) \\ u(t) = \nu_c(t)$
  note: $I.C. := \nu(0)$
  note: $\nu_c(t)$
  note: $\nu(t)$
  In1 nu_c : Inport
  I.C. = nu(0) : StateSpace  A=-pnu  B=pnu  D=0  InitialCondition=nu0
  Out1 nu : Outport
  wires:
  In1 nu_c/1 -> I.C. = nu(0)/1
  I.C. = nu(0)/1 -> Out1 nu/1

== system nape_speed_brakes/Thrust Cont. Law/I.C.=T(0) ==
  note: $T_c(t)$
  note: $x(t) = T(t) \\ u(t) = T_c(t)$
  note: $I.C. := T(0)$
  note: $T(t)$
  In1 Tc(t) : Inport
  I.C.=T(0) : StateSpace  A=-pT  B=pT  D=0  InitialCondition=T0
  Out1 T(t) : Outport
  wires:
  In1 Tc(t)/1 -> I.C.=T(0)/1
  I.C.=T(0)/1 -> Out1 T(t)/1

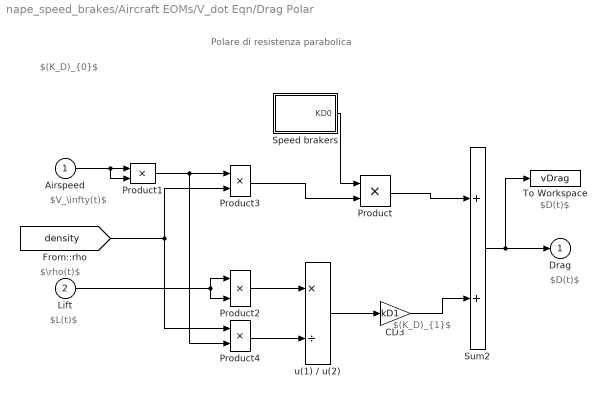
== system nape_speed_brakes/Aircraft EOMs/V_dot Eqn/Drag Polar ==
  note: Polare di resistenza parabolica
  note: $V_\infty(t)$
  note: $L(t)$
  note: $(K_D)_{1}$
  note: $D(t)$
  note: $D(t)$
  note: $\rho(t)$
  note: $(K_D)_{0}$
  Airspeed : Inport
  Lift : Inport  Port=2
  CD3 : Gain  Gain=kD1  SaturateOnIntegerOverflow=on  OutDataTypeStr=Inherit: Same as input  ParamDataTypeStr=Inherit: Same as input
  Product : Product
  Product{1..4} (4 alike) : Product  InputSameDT=on  RndMeth=Zero  SaturateOnIntegerOverflow=on  OutDataTypeStr=Inherit: Same as first input
  Speed brakers : Subsystem
  Sum2 : Sum  InputSameDT=on  SaturateOnIntegerOverflow=on  OutDataTypeStr=Inherit: Same as first input
  To Workspace : ToWorkspace  VariableName=vDrag  SaveFormat=Timeseries
  u(1) / u(2) : Product  Inputs=*/
  Drag : Outport
  wires:
  Lift/1 -> Product2/1, Product2/2
  Airspeed/1 -> Product1/2, Product1/1
  Product1/1 -> Product4/2, Product3/1
  Sum2/1 -> To Workspace/1, Drag/1
  [density] -> Product3/2, Product4/1
  Product2/1 -> u(1) / u(2)/1
  u(1) / u(2)/1 -> CD3/1
  Product4/1 -> u(1) / u(2)/2
  CD3/1 -> Sum2/2
  Product3/1 -> Product/2
  Product/1 -> Sum2/1
  Speed brakers/1(KD0) -> Product/1

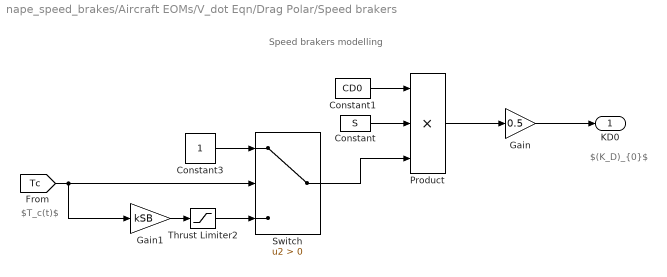
== system nape_speed_brakes/Aircraft EOMs/V_dot Eqn/Drag Polar/Speed brakers ==
  note: $T_c(t)$
  note: $(K_D)_{0}$
  note: Speed brakers modelling
  Constant : Constant  Value=S
  Constant1 : Constant  Value=CD0
  Constant3 : Constant
  Gain : Gain  Gain=0.5
  Gain1 : Gain  Gain=kSB
  Product : Product  Inputs=3
  Switch : Switch  Criteria=u2 > Threshold  SaturateOnIntegerOverflow=off  InputSameDT=off
  Thrust Limiter2 : Saturate  UpperLimit=SB_DragFactorMax  LowerLimit=1
  KD0 : Outport
  wires:
  Gain1/1 -> Thrust Limiter2/1
  Thrust Limiter2/1 -> Switch/3
  Constant3/1 -> Switch/1
  [Tc] -> Switch/2, Gain1/1
  Gain/1 -> KD0/1
  Switch/1 -> Product/3
  Product/1 -> Gain/1
  Constant/1 -> Product/2
  Constant1/1 -> Product/1
